simulink model "DC_Bazen_Externe_Merania_v08_SK"  (R2026a)
settings: Solver=FixedStepDiscrete  StopTime=603900  FixedStep=900
settings Model: Creator=Lysda  LastModifiedBy=Lysda

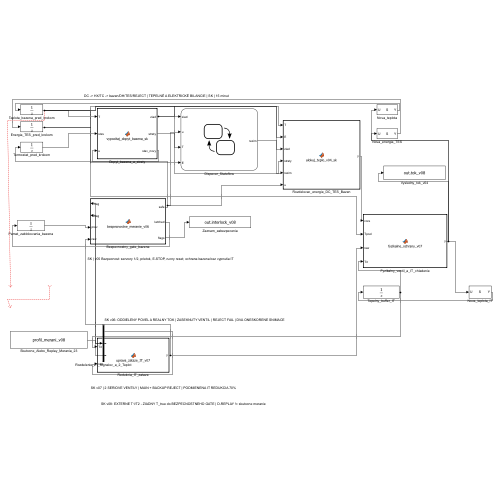
[thumbnail: Simulink's stored preview of the top-level diagram]
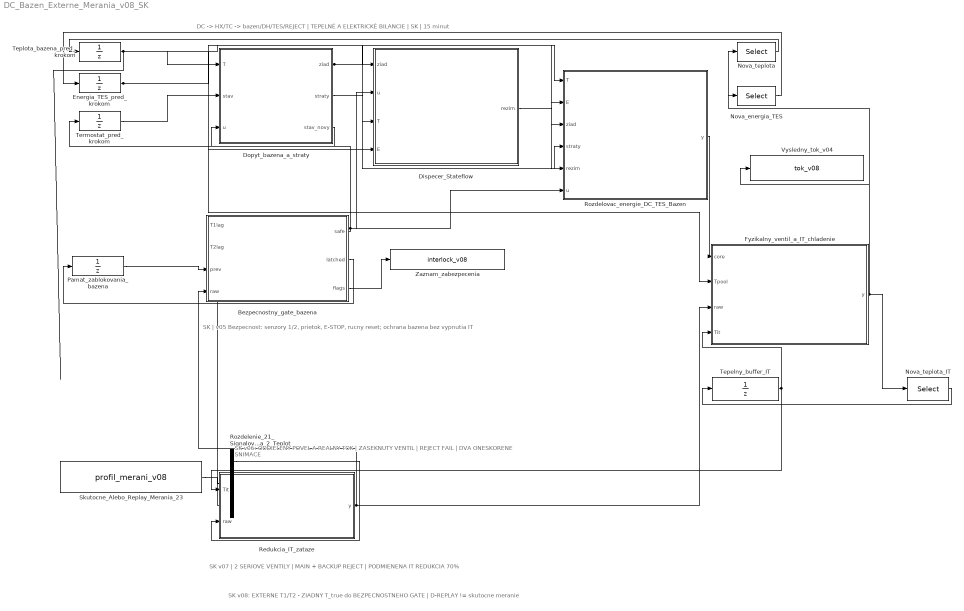
== system DC_Bazen_Externe_Merania_v08_SK ==
  note: DC -> HX/TC -> bazen/DH/TES/REJECT | TEPELNÉ A ELEKTRICKÉ BILANCIE | SK | 15 minut
  note: SK | v05 Bezpecnost: senzory 1/2, prietok, E-STOP, rucny reset; ochrana bazena bez vypnutia IT
  note: SK v06: ODDIELENY POVEL A REALNY TOK | ZASEKNUTY VENTIL | REJECT FAIL | DVA ONESKORENE SNIMACE
  note: SK v07 | 2 SERIOVE VENTILY | MAIN + BACKUP REJECT | PODMIENENA IT REDUKCIA 70%
  note: SK v08: EXTERNE T1/T2 - ZIADNY T_true do BEZPECNOSTNEHO GATE | D-REPLAY != skutocne meranie
  Bezpecnostny_gate_bazena : MATLAB Function  TreatAsAtomicUnit=on
  Dispecer_Stateflow : Stateflow chart  TreatAsAtomicUnit=on
  Dopyt_bazena_a_straty : MATLAB Function  TreatAsAtomicUnit=on
  Energia_TES_pred_krokom : UnitDelay  InitialCondition=0.45*3.6e9  SampleTime=900
  Fyzikalny_ventil_a_IT_chladenie : MATLAB Function  TreatAsAtomicUnit=on
  Nova_energia_TES : Selector  InputPortWidth=39  IndexOptions=Index vector (dialog)  Indices=2  OutputSizes=1
  Nova_teplota : Selector  InputPortWidth=39  IndexOptions=Index vector (dialog)  Indices=1  OutputSizes=1
  Nova_teplota_IT : Selector  InputPortWidth=39  IndexOptions=Index vector (dialog)  Indices=28  OutputSizes=1
  Pamat_zablokovania_bazena : UnitDelay  SampleTime=900
  Redukcia_IT_zataze : MATLAB Function  TreatAsAtomicUnit=on
  Rozdelenie_21_Signalov_a_2_Teplot : Demux  Outputs=[21 1 1]
  Rozdelovac_energie_DC_TES_Bazen : MATLAB Function  TreatAsAtomicUnit=on
  Skutocne_Alebo_Replay_Merania_23 : FromWorkspace  VariableName=profil_merani_v08  OutputAfterFinalValue=Holding final value
  Tepelny_buffer_IT : UnitDelay  InitialCondition=30  SampleTime=900
  Teplota_bazena_pred_krokom : UnitDelay  InitialCondition=16  SampleTime=900
  Termostat_pred_krokom : UnitDelay  InitialCondition=1  SampleTime=900
  Vysledny_tok_v04 : ToWorkspace  VariableName=tok_v08  SaveFormat=Timeseries  SampleTime=-1
  Zaznam_zabezpecenia : ToWorkspace  VariableName=interlock_v08  SaveFormat=Timeseries  SampleTime=-1
  wires:
  Teplota_bazena_pred_krokom/1 -> Dopyt_bazena_a_straty/1(T), Dispecer_Stateflow/3(T), Rozdelovac_energie_DC_TES_Bazen/1(T), Fyzikalny_ventil_a_IT_chladenie/2(Tpool)
  Termostat_pred_krokom/1 -> Dopyt_bazena_a_straty/2(stav)
  Dopyt_bazena_a_straty/3(stav_novy) -> Termostat_pred_krokom/1
  Dopyt_bazena_a_straty/1(ziad) -> Dispecer_Stateflow/1(ziad), Rozdelovac_energie_DC_TES_Bazen/3(ziad)
  Energia_TES_pred_krokom/1 -> Dispecer_Stateflow/4(E), Rozdelovac_energie_DC_TES_Bazen/2(E)
  Dopyt_bazena_a_straty/2(straty) -> Rozdelovac_energie_DC_TES_Bazen/4(straty)
  Dispecer_Stateflow/1(rezim) -> Rozdelovac_energie_DC_TES_Bazen/5(rezim)
  Nova_teplota/1 -> Teplota_bazena_pred_krokom/1
  Nova_energia_TES/1 -> Energia_TES_pred_krokom/1
  Bezpecnostny_gate_bazena/2(latched) -> Pamat_zablokovania_bazena/1
  Bezpecnostny_gate_bazena/3(flags) -> Zaznam_zabezpecenia/1
  Bezpecnostny_gate_bazena/1(safe) -> Dopyt_bazena_a_straty/3(u), Dispecer_Stateflow/2(u), Rozdelovac_energie_DC_TES_Bazen/6(u)
  ? -> ?
  Pamat_zablokovania_bazena/1 -> Bezpecnostny_gate_bazena/3(prev)
  Rozdelovac_energie_DC_TES_Bazen/1(y) -> Fyzikalny_ventil_a_IT_chladenie/1(core)
  Tepelny_buffer_IT/1 -> Fyzikalny_ventil_a_IT_chladenie/4(Tit), Redukcia_IT_zataze/1(Tit)
  Fyzikalny_ventil_a_IT_chladenie/1(y) -> Nova_teplota/1, Nova_energia_TES/1, Vysledny_tok_v04/1, Nova_teplota_IT/1
  Nova_teplota_IT/1 -> Tepelny_buffer_IT/1
  Redukcia_IT_zataze/1(y) -> Bezpecnostny_gate_bazena/4(raw), Fyzikalny_ventil_a_IT_chladenie/3(raw)
  Skutocne_Alebo_Replay_Merania_23/1 -> Rozdelenie_21_Signalov_a_2_Teplot/1
  Rozdelenie_21_Signalov_a_2_Teplot/1 -> Redukcia_IT_zataze/2(raw)
  Rozdelenie_21_Signalov_a_2_Teplot/2 -> Bezpecnostny_gate_bazena/1(T1lag)
  Rozdelenie_21_Signalov_a_2_Teplot/3 -> Bezpecnostny_gate_bazena/2(T2lag)

== matlab function DC_Bazen_Externe_Merania_v08_SK/Bezpecnostny_gate_bazena ==
  data: T1lag input; safe output size=[1 11]; T2lag input; prev input; raw input size=[1 22]; latched output; flags output size=[1 10]
function [safe,latched,flags] = bezpecnostne_meranie_v06(T1lag,T2lag,prev,raw)
%#codegen
% v08: T1lag/T2lag = EXTERNE kalibrovane meracie hodnoty s uz aplikovanym
% bias/senzorickym oneskorenim. NEVER add raw(12/13) again!
% raw 1:11 BMS, 14 flowOK, 15 ESTOP, 16 manual reset.
safe=zeros(1,11);
for k=1:11,safe(k)=raw(k);end
t1=T1lag;t2=T2lag;
valid=isfinite(t1)&&isfinite(t2);
mismatch=valid&&(abs(t1-t2)>0.35);
hot=valid&&((t1>=27.70)||(t2>=27.70));
flowFault=raw(14)<0.5;
estop=raw(15)>0.5;
fault=(~valid)||mismatch||hot||flowFault||estop;
latched=double(prev>0.5);
resetOK=0;
if fault
    latched=1;
elseif raw(16)>0.5 && latched>0.5 && max(t1,t2)<=27.65
    latched=0;resetOK=1;
end
if latched>0.5,safe(9)=0;end
flags=zeros(1,10);
flags(1)=latched;flags(2)=double(mismatch);
flags(3)=double(hot);flags(4)=double(flowFault);
flags(5)=double(estop);flags(6)=double(~valid);
flags(7)=resetOK;flags(8)=t1;flags(9)=t2;
flags(10)=safe(9);
end

== matlab function DC_Bazen_Externe_Merania_v08_SK/Fyzikalny_ventil_a_IT_chladenie ==
  data: core input size=[1 25]; y output size=[1 39]; Tpool input; raw input size=[1 22]; Tit input
function y=fyzikalne_ochrany_v07(core,Tpool,raw,Tit)
%#codegen
% Separatne dve uzatvaracie vetvy HX: fyzicky unik len pri dvoch poruchach.
% REJECT A =180 kW, REJECT B=150 kW; oba su scenarove hodnoty.
% raw 17 primary stuck, 19 secondary stuck, 18 main reject availability,
% 20 backup reject availability. raw 22 = Q_IT_load_avoided (W).
dt=900; Cw=997*500*4182; Cit=8e6;
Qcmd=max(0,core(4));
QrejectCmd=max(0,core(17));
Qdc=max(0,core(18));
primaryFault=raw(17)>0.5;
backupFault=raw(19)>0.5;
leak=0;
if primaryFault && backupFault && Qcmd<=1e-7
    drive=max(0,raw(2)-Tpool-3);
    leak=min([25000,QrejectCmd,4500*drive]);
end
Qremaining=max(0,QrejectCmd-leak);
mainCap=180000*min(1,max(0,raw(18)));
backupCap=150000*min(1,max(0,raw(20)));
QrejectA=min(Qremaining,mainCap);
QrejectB=min(max(0,Qremaining-QrejectA),backupCap);
Qreject=QrejectA+QrejectB;
Qunhandled=max(0,Qremaining-Qreject);
passive=max(0,2000*(Tit-30));
TitNext=max(30,Tit+dt*(Qunhandled-passive)/Cit);
y=zeros(1,39);
for k=1:25,y(k)=core(k);end
y(1)=core(1)+dt*leak/Cw;
y(4)=Qcmd+leak;
y(6)=core(6)+leak;
y(17)=Qreject;
% Include accumulated, not-dissipated heat explicitly in closure
y(22)=Qdc-(y(6)+core(14)+Qreject+Qunhandled);
y(24)=y(4)-(y(6)+core(7));
y(26)=leak;
y(27)=Qunhandled;
y(28)=TitNext;
y(29)=double(TitNext>=42); 
y(30)=QrejectCmd;
y(31)=Qreject;
y(32)=double((Qcmd<=1e-7)&&(leak>0));
y(33)=y(22);
y(34)=QrejectA;
y(35)=QrejectB;
y(36)=max(0,raw(22)); % avoided modeled waste heat
y(37)=double(primaryFault);
y(38)=double(backupFault);
y(39)=Qremaining-(QrejectA+QrejectB+Qunhandled);
end

== matlab function DC_Bazen_Externe_Merania_v08_SK/Redukcia_IT_zataze ==
  data: Tit input; y output size=[1 22]; raw input size=[1 21]
function y=uprava_zataze_IT_v07(Tit,raw)
%#codegen
% Nova ochrana; redukcia zataze IT pri strate OBOCH chladiacich vetiev.
% 21 vstupov, Q_DC je dostupne odpadove teplo [W], nie elektricka energia.
% 21: povolena automaticka redukcia IT zataze [0/1].
y=zeros(1,22);
for k=1:21
    y(k)=raw(k);
end
shed=0;
if (raw(18)<0.5) && (raw(20)<0.5) && raw(21)>0.5 && Tit>=38
    shed=0.70*max(0,raw(1)); % scenarovy okamzity pokles o 70%
    y(1)=max(0,raw(1)-shed);
end
y(22)=shed;
end

== matlab function DC_Bazen_Externe_Merania_v08_SK/Rozdelovac_energie_DC_TES_Bazen ==
  data: T input; E input; ziad input; straty input; rezim input; u input size=[1 11]; y output size=[1 25]
function y = alokuj_teplo_v04_sk(T,E,ziad,straty,rezim,u)
%#codegen
% Stav T [C], energia TES E[J], ziad/straty [W], rezim Stateflow 0..4.
% Tepelny zdroj DC: len skutocne dostupny tok, nikdy IT nominal.
dt=900; C=997*500*4182;
Emax=900*3.6e6; % 900 kWh
eta_c=0.93; eta_d=0.91;
Qdc=max(0,u(1)); Tdc=u(2); Qdhneed=max(0,u(3));
TES_ok=u(10)>0.5;
Qtesloss=0.002*max(0,E)/86400;
Qdirect=0; QhpPool=0; QhpDH=0; Qcharge=0; Qdis=0;
QhpSrc=0; Pel=0; Paux=0; cop=0;
if (rezim==1) && u(11)>0.5 && u(9)>0.5
    % 5 K approach; konduktancia je predpoklad, nie navrh doskoveho HX.
    Qhxmax=max(0,8500*(Tdc-T-5));
    Qdirect=min([ziad,Qdc,150000,Qhxmax]);
end
Qleft=max(0,Qdc-Qdirect);
if rezim==1 || rezim==2
    % T kondenzatora 52 C, T vyparnika Tdc-5 C; Carnot * 0.43.
    % Bez manufacturer COP(Tsource,Tsink,PLR) = iba scenar.
    Tevap=Tdc-5; Tcond=52;
    cop=min(6,max(2.5,0.43*(Tcond+273.15)/max(5,Tcond-Tevap)));
    QhpCap=min([200000,55000*cop,Qleft/max(1e-9,1-1/cop)]);
    % Minimalna priorita tepelnej siete: rezervuj max 50 kW.
    minDH=min(Qdhneed,min(50000,QhpCap));
    QhpPool=min(max(0,ziad-Qdirect),max(0,QhpCap-minDH));
    QhpDH=min(Qdhneed,QhpCap-QhpPool);
    spare=max(0,QhpCap-QhpPool-QhpDH);
    extraPool=min(max(0,ziad-Qdirect-QhpPool),spare);
    QhpPool=QhpPool+extraPool;
    spare=max(0,QhpCap-QhpPool-QhpDH);
    % Nabijame TES az po aktualnom bazene a obsluhe siete.
    if TES_ok && E<Emax && spare>0
        room=max(0,(Emax-E+Qtesloss*dt)/(eta_c*dt));
        Qcharge=min([spare,70000,room]);
    end
    QhpOut=QhpPool+QhpDH+Qcharge;
    Pel=QhpOut/cop;
    QhpSrc=QhpOut-Pel;
    if QhpOut>0,Paux=1500;end
end
if Qdirect>0,Paux=Paux+500;end
Qpool=Qdirect+QhpPool;
QdhShort=max(0,Qdhneed-QhpDH);
if TES_ok && QdhShort>0 && E>0
    transferable=max(0,(E-Qtesloss*dt)*eta_d/dt);
    Qdis=min([QdhShort,80000,transferable]);
    if Qdis>0,Paux=Paux+250;end
end
% TES nesmie sucasne nabijat a vybijat.
if Qdis>0 && Qcharge>0
    Qcharge=0;
    QhpOut=QhpPool+QhpDH;
    Pel=QhpOut/cop;
    QhpSrc=QhpOut-Pel;
end
Qdh=QhpDH+Qdis;
Qreject=max(0,Qdc-Qdirect-QhpSrc);
Enext=max(0,min(Emax,E+dt*(eta_c*Qcharge-Qdis/eta_d-Qtesloss)));
Tnext=T+dt*(Qpool-straty)/C;
qsourceResidual=Qdc-(Qdirect+QhpSrc+Qreject);
qhpResidual=(QhpPool+QhpDH+Qcharge)-(QhpSrc+Pel);
qpoolResidual=Qpool-(Qdirect+QhpPool);
qdhResidual=Qdh-(QhpDH+Qdis);
y=zeros(1,25);
y(1)=Tnext;
y(2)=Enext;
y(3)=ziad;
y(4)=Qpool;
y(5)=straty;
y(6)=Qdirect;
y(7)=QhpPool;
y(8)=QhpDH;
y(9)=Qcharge;
y(10)=Qdis;
y(11)=Qdh;
y(12)=max(0,Qdhneed-Qdh);
y(13)=max(0,ziad-Qpool);
y(14)=QhpSrc;
y(15)=Pel;
y(16)=Paux;
y(17)=Qreject;
y(18)=Qdc;
y(19)=cop;
y(20)=rezim;
y(21)=Qtesloss;
y(22)=qsourceResidual;
y(23)=qhpResidual;
y(24)=qpoolResidual;
y(25)=qdhResidual;
end

== matlab function DC_Bazen_Externe_Merania_v08_SK/Dopyt_bazena_a_straty ==
  data: T input; stav input; u input size=[1 11]; ziad output; straty output; stav_novy output
function [ziad,straty,stav_novy] = vypocitaj_dopyt_bazena_sk(T,stav,u)
%#codegen
% u [Qdc_W,Tdc_C,Qdh_W,Tair_C,RH,aktivita,plachta,IT_ok,BAZEN_ok,TES_ok,HX_ok].
% Vykony W, teploty C, krok 900 s, objem 500 m3.
A=312.5; C=997*500*4182; dt=900; cp=4182;
Ta=u(4);rh=min(1,max(0,u(5)));
activity=max(0,u(6));cover=min(1,max(0,u(7)));
pv=0.61094*exp(17.625*T/(T+243.04));
pa=rh*0.61094*exp(17.625*Ta/(Ta+243.04));
mv=max(0,4e-5*A*(pv-pa)*activity*(1-0.9*cover));
Qevap=mv*2440000;
Qconv=3*A*(T-Ta)*(1-0.75*cover);
Qrad=0.95*5.670374419e-8*A*((T+273.15)^4-(Ta-2+273.15)^4)*(1-0.75*cover);
Qkonstr=800*(T-20);
Qmakeup=mv*cp*(T-15);
straty=Qevap+Qconv+Qrad+Qkonstr+Qmakeup+2000;
stav_novy=stav;
if T<=27.35,stav_novy=1;elseif T>=27.65,stav_novy=0;end
if u(9)<0.5
    stav_novy=0;
end
ziad=0;
if stav_novy>0.5 && T<27.75 && u(9)>0.5
    Qsafe=max(0,(27.75-T)*C/dt+straty);
    Qset=max(0,(27.58-T)*C/dt+straty);
    ziad=min([150000,Qsafe,Qset]);
end
end

== stateflow chart DC_Bazen_Externe_Merania_v08_SK/Dispecer_Stateflow ==
  settings: updateMethod=DISCRETE  sampleTime=900  description=Stavy dispecera su realne Stateflow; ich prechody zavisia od teploty bazena, jeho dopytu, zdroja a TES.
  state BEZ_ZDROJA
    en,du:
    rezim=0;
  state PRIAMY_VYMENNIK
    en,du:
    rezim=1;
  state TEPELNE_CERPADLO
    en,du:
    rezim=2;
  state CERPAJ_Z_TES
    en,du:
    rezim=3;
  state IT_BEZPECNE_ODSTAVENIE
    en,du:
    rezim=4;
  (junction 17) -> TEPELNE_CERPADLO [order 3] : [volba_rezimu_v04_sk(ziad,u,T,E)==2]
  (default) -> (junction 17)
  (junction 17) -> PRIAMY_VYMENNIK [order 2] : [volba_rezimu_v04_sk(ziad,u,T,E)==1]
  (junction 17) -> BEZ_ZDROJA [order 1] : [volba_rezimu_v04_sk(ziad,u,T,E)==0]
  (junction 17) -> CERPAJ_Z_TES [order 4] : [volba_rezimu_v04_sk(ziad,u,T,E)==3]
  (junction 17) -> IT_BEZPECNE_ODSTAVENIE [order 5] : [volba_rezimu_v04_sk(ziad,u,T,E)==4]
  TEPELNE_CERPADLO -> CERPAJ_Z_TES [order 3] : [volba_rezimu_v04_sk(ziad,u,T,E)==3]
  PRIAMY_VYMENNIK -> CERPAJ_Z_TES [order 3] : [volba_rezimu_v04_sk(ziad,u,T,E)==3]
  TEPELNE_CERPADLO -> IT_BEZPECNE_ODSTAVENIE [order 4] : [volba_rezimu_v04_sk(ziad,u,T,E)==4]
  TEPELNE_CERPADLO -> BEZ_ZDROJA [order 1] : [volba_rezimu_v04_sk(ziad,u,T,E)==0]
  CERPAJ_Z_TES -> BEZ_ZDROJA [order 1] : [volba_rezimu_v04_sk(ziad,u,T,E)==0]
  IT_BEZPECNE_ODSTAVENIE -> BEZ_ZDROJA [order 1] : [volba_rezimu_v04_sk(ziad,u,T,E)==0]
  PRIAMY_VYMENNIK -> BEZ_ZDROJA [order 1] : [volba_rezimu_v04_sk(ziad,u,T,E)==0]
  CERPAJ_Z_TES -> PRIAMY_VYMENNIK [order 2] : [volba_rezimu_v04_sk(ziad,u,T,E)==1]
  CERPAJ_Z_TES -> TEPELNE_CERPADLO [order 3] : [volba_rezimu_v04_sk(ziad,u,T,E)==2]
  IT_BEZPECNE_ODSTAVENIE -> PRIAMY_VYMENNIK [order 2] : [volba_rezimu_v04_sk(ziad,u,T,E)==1]
  BEZ_ZDROJA -> PRIAMY_VYMENNIK [order 1] : [volba_rezimu_v04_sk(ziad,u,T,E)==1]
  BEZ_ZDROJA -> TEPELNE_CERPADLO [order 2] : [volba_rezimu_v04_sk(ziad,u,T,E)==2]
  TEPELNE_CERPADLO -> PRIAMY_VYMENNIK [order 2] : [volba_rezimu_v04_sk(ziad,u,T,E)==1]
  IT_BEZPECNE_ODSTAVENIE -> TEPELNE_CERPADLO [order 3] : [volba_rezimu_v04_sk(ziad,u,T,E)==2]
  PRIAMY_VYMENNIK -> TEPELNE_CERPADLO [order 2] : [volba_rezimu_v04_sk(ziad,u,T,E)==2]
  BEZ_ZDROJA -> CERPAJ_Z_TES [order 3] : [volba_rezimu_v04_sk(ziad,u,T,E)==3]
  PRIAMY_VYMENNIK -> IT_BEZPECNE_ODSTAVENIE [order 4] : [volba_rezimu_v04_sk(ziad,u,T,E)==4]
  BEZ_ZDROJA -> IT_BEZPECNE_ODSTAVENIE [order 4] : [volba_rezimu_v04_sk(ziad,u,T,E)==4]
  IT_BEZPECNE_ODSTAVENIE -> CERPAJ_Z_TES [order 4] : [volba_rezimu_v04_sk(ziad,u,T,E)==3]
  CERPAJ_Z_TES -> IT_BEZPECNE_ODSTAVENIE [order 4] : [volba_rezimu_v04_sk(ziad,u,T,E)==4]
  data: req function_input; inputs function_input; waterTemperature function_input; storedEnergy function_input; m function_output; ziad input size=1; u input size=[1 11]; T input size=1; E input size=1; rezim output size=1
  function m=volba_rezimu_v04_sk(req,inputs,waterTemperature,storedEnergy):
    | function m=volba_rezimu_v04_sk(req,inputs,waterTemperature,storedEnergy)
    | % Opravena lokálna symbolika funkcie Stateflow, bez tienovania chart dat.
    | m=0;
    | if inputs(8)<0.5
    |     m=4; % IT zastavene
    | elseif inputs(1)<=1e-6
    |     if storedEnergy>100000 && inputs(10)>0.5 && inputs(3)>0
    |         m=3; % TES-only
    |     end
    | elseif inputs(11)>0.5 && inputs(9)>0.5 && req>0 && inputs(2)>waterTemperature+5
    |     m=1; % priamy HX bazena, TC sluzba siete
    | else
    |     m=2; % TC
    | end
    | end
